simulink model "chap_FIS"  (R2024b)
settings: Solver=VariableStepAuto  StartTime=0.0  StopTime=10.0  RelTol=1e-3
libraries: fuzblock x1
settings Model: Creator=33242  LastModifiedBy=33242

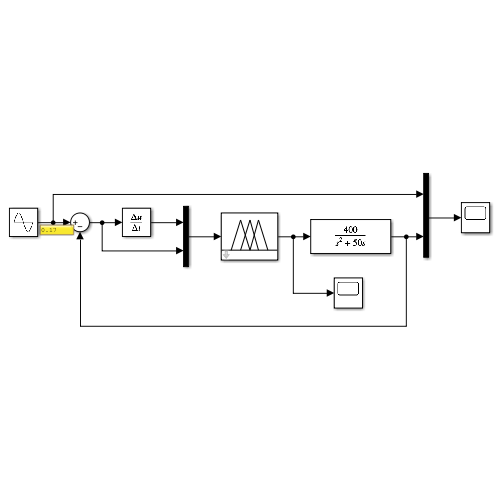
[thumbnail: Simulink's stored preview of the top-level diagram]
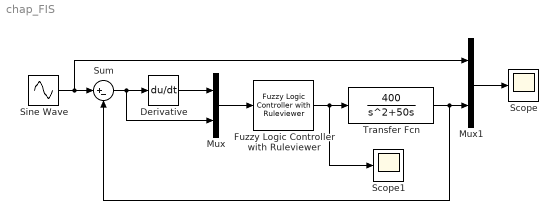
== system chap_FIS ==
  Derivative : Derivative
  Fuzzy Logic Controller with Ruleviewer : fuzblock/Fuzzy Logic  Controller  with Ruleviewer  fismatrix=a2  Ts=2
  Mux : Mux  Inputs=2
  Mux1 : Mux  Inputs=2
  Scope : Scope
  Scope1 : Scope
  Sine Wave : Sin  Amplitude=0.5  Frequency=10  SampleTime=0
  Sum : Sum  Inputs=|+-
  Transfer Fcn : TransferFcn  Numerator=[400]  Denominator=[1 50 0]
  wires:
  Fuzzy Logic Controller with Ruleviewer/1 -> Scope1/1, Transfer Fcn/1
  Sine Wave/1 -> Mux1/1, Sum/1
  Sum/1 -> Derivative/1, Mux/2
  Derivative/1 -> Mux/1
  Mux/1 -> Fuzzy Logic Controller with Ruleviewer/1
  Transfer Fcn/1 -> Sum/2, Mux1/2
  Mux1/1 -> Scope/1
